simulink model "Takahashi1986_DTC"  (R2024b)
settings: Solver=FixedStepDiscrete  StartTime=0.0  StopTime=.62  FixedStep=Ts  RelTol=1e-3
InitFcn:
  | demoModel=bdroot; demoWorkspace=get_param(demoModel,'ModelWorkspace');
  | demoCases=getVariable(demoWorkspace,'DemoCases');
  | demoCaseName=get_param([demoModel '/Experiment_Settings'],'CaseName');
  | demoSelected=find(strcmp(demoCaseName,{demoCases.name}),1);
  | demoValues=demoCases(demoSelected).variables; demoNames=fieldnames(demoValues);
  | for demoIndex=1:numel(demoNames), assignin(demoWorkspace,demoNames{demoIndex},demoValues.(demoNames{demoIndex})); end
  | clear demoModel demoWorkspace demoCases demoCaseName demoSelected demoValues demoNames demoIndex;
model workspace (MAT data in the model file):
  DemoCases(1).name = 'Wide_band_0p40Nm'
  DemoCases(1).variables.ScenarioInput{1} = timeseries
  DemoCases(1).variables.ScenarioInput{1}.Name = 'unnamed'
  DemoCases(1).variables.ScenarioInput{1}.DataInfo = tsdata.datametadata
  DemoCases(1).variables.ScenarioInput{1}.DataInfo.Interpolation = tsdata.interpolation
  DemoCases(1).variables.ScenarioInput{1}.DataInfo.Interpolation.Fhandle : function handle (value not decoded)
  DemoCases(1).variables.ScenarioInput{1}.DataInfo.Interpolation.Name = 'linear'
  DemoCases(1).variables.ScenarioInput{1}.TimeInfo = tsdata.timemetadata
  DemoCases(1).variables.ScenarioInput{1}.TimeInfo.Length = 24801
  DemoCases(1).variables.ScenarioInput{1}.TimeInfo.DuplicateTimes = 0
  DemoCases(1).variables.ScenarioInput{1}.TimeInfo.Time_ = [0 2.5e-05 5e-05 7.5e-05 0.0001 0.000125 0.00015 0.000175 0.0002 0.000225 0.00025 0.000275 ... (24801 elements, 24801x1)]
  DemoCases(1).variables.ScenarioInput{1}.TimeInfo.Initialized = 1
  DemoCases(1).variables.ScenarioInput{1}.QualityInfo = tsdata.qualmetadata
  DemoCases(1).variables.ScenarioInput{1}.Data_ = [0.419999986887 0.419999986887 0.419999986887 0.419999986887 0.419999986887 0.419999986887 0.419999986887 0.419999986887 0.419999986887 0.419999986887 0.419999986887 0.419999986887 ... (24801 elements, 24801x1)]
  DemoCases(1).variables.ScenarioInput{2} = timeseries
  DemoCases(1).variables.ScenarioInput{2}.Name = 'unnamed'
  DemoCases(1).variables.ScenarioInput{2}.DataInfo = tsdata.datametadata
  DemoCases(1).variables.ScenarioInput{2}.DataInfo.Interpolation = tsdata.interpolation
  DemoCases(1).variables.ScenarioInput{2}.DataInfo.Interpolation.Fhandle : function handle (value not decoded)
  DemoCases(1).variables.ScenarioInput{2}.DataInfo.Interpolation.Name = 'linear'
  DemoCases(1).variables.ScenarioInput{2}.TimeInfo = tsdata.timemetadata
  DemoCases(1).variables.ScenarioInput{2}.TimeInfo.Length = 24801
  DemoCases(1).variables.ScenarioInput{2}.TimeInfo.DuplicateTimes = 0
  DemoCases(1).variables.ScenarioInput{2}.TimeInfo.Time_ = [0 2.5e-05 5e-05 7.5e-05 0.0001 0.000125 0.00015 0.000175 0.0002 0.000225 0.00025 0.000275 ... (24801 elements, 24801x1)]
  DemoCases(1).variables.ScenarioInput{2}.TimeInfo.Initialized = 1
  DemoCases(1).variables.ScenarioInput{2}.QualityInfo = tsdata.qualmetadata
  DemoCases(1).variables.ScenarioInput{2}.Data_ = [0 0 0 0 0 0 0 0 0 0 0 0 ... (24801 elements, 24801x1)]
  DemoCases(1).variables.ScenarioInput{3} = timeseries
  DemoCases(1).variables.ScenarioInput{3}.Name = 'unnamed'
  DemoCases(1).variables.ScenarioInput{3}.DataInfo = tsdata.datametadata
  DemoCases(1).variables.ScenarioInput{3}.DataInfo.Interpolation = tsdata.interpolation
  DemoCases(1).variables.ScenarioInput{3}.DataInfo.Interpolation.Fhandle : function handle (value not decoded)
  DemoCases(1).variables.ScenarioInput{3}.DataInfo.Interpolation.Name = 'linear'
  DemoCases(1).variables.ScenarioInput{3}.TimeInfo = tsdata.timemetadata
  DemoCases(1).variables.ScenarioInput{3}.TimeInfo.Length = 24801
  DemoCases(1).variables.ScenarioInput{3}.TimeInfo.DuplicateTimes = 0
  DemoCases(1).variables.ScenarioInput{3}.TimeInfo.Time_ = [0 2.5e-05 5e-05 7.5e-05 0.0001 0.000125 0.00015 0.000175 0.0002 0.000225 0.00025 0.000275 ... (24801 elements, 24801x1)]
  DemoCases(1).variables.ScenarioInput{3}.TimeInfo.Initialized = 1
  DemoCases(1).variables.ScenarioInput{3}.QualityInfo = tsdata.qualmetadata
  DemoCases(1).variables.ScenarioInput{3}.Data_ = [0.40000000596 0.40000000596 0.40000000596 0.40000000596 0.40000000596 0.40000000596 0.40000000596 0.40000000596 0.40000000596 0.40000000596 0.40000000596 0.40000000596 ... (24801 elements, 24801x1)]
  DemoCases(1).variables.ScenarioInput{4} = timeseries
  DemoCases(1).variables.ScenarioInput{4}.Name = 'unnamed'
  DemoCases(1).variables.ScenarioInput{4}.DataInfo = tsdata.datametadata
  DemoCases(1).variables.ScenarioInput{4}.DataInfo.Interpolation = tsdata.interpolation
  DemoCases(1).variables.ScenarioInput{4}.DataInfo.Interpolation.Fhandle : function handle (value not decoded)
  DemoCases(1).variables.ScenarioInput{4}.DataInfo.Interpolation.Name = 'linear'
  DemoCases(1).variables.ScenarioInput{4}.TimeInfo = tsdata.timemetadata
  DemoCases(1).variables.ScenarioInput{4}.TimeInfo.Length = 24801
  DemoCases(1).variables.ScenarioInput{4}.TimeInfo.DuplicateTimes = 0
  DemoCases(1).variables.ScenarioInput{4}.TimeInfo.Time_ = [0 2.5e-05 5e-05 7.5e-05 0.0001 0.000125 0.00015 0.000175 0.0002 0.000225 0.00025 0.000275 ... (24801 elements, 24801x1)]
  DemoCases(1).variables.ScenarioInput{4}.TimeInfo.Initialized = 1
  DemoCases(1).variables.ScenarioInput{4}.QualityInfo = tsdata.qualmetadata
  DemoCases(1).variables.ScenarioInput{4}.Data_ = [100 100 100 100 100 100 100 100 100 100 100 100 ... (24801 elements, 24801x1)]
  DemoCases(1).variables.ScenarioInput{5} = timeseries
  DemoCases(1).variables.ScenarioInput{5}.Name = 'unnamed'
  DemoCases(1).variables.ScenarioInput{5}.DataInfo = tsdata.datametadata
  DemoCases(1).variables.ScenarioInput{5}.DataInfo.Interpolation = tsdata.interpolation
  DemoCases(1).variables.ScenarioInput{5}.DataInfo.Interpolation.Fhandle : function handle (value not decoded)
  DemoCases(1).variables.ScenarioInput{5}.DataInfo.Interpolation.Name = 'linear'
  DemoCases(1).variables.ScenarioInput{5}.TimeInfo = tsdata.timemetadata
  DemoCases(1).variables.ScenarioInput{5}.TimeInfo.Length = 24801
  DemoCases(1).variables.ScenarioInput{5}.TimeInfo.DuplicateTimes = 0
  DemoCases(1).variables.ScenarioInput{5}.TimeInfo.Time_ = [0 2.5e-05 5e-05 7.5e-05 0.0001 0.000125 0.00015 0.000175 0.0002 0.000225 0.00025 0.000275 ... (24801 elements, 24801x1)]
  DemoCases(1).variables.ScenarioInput{5}.TimeInfo.Initialized = 1
  DemoCases(1).variables.ScenarioInput{5}.QualityInfo = tsdata.qualmetadata
  DemoCases(1).variables.ScenarioInput{5}.Data_ = [0 0 0 0 0 0 0 0 0 0 0 0 ... (24801 elements, 24801x1)]
  DemoCases(2).name = 'Narrow_band_0p15Nm'
  DemoCases(2).variables.ScenarioInput{1} = timeseries
  DemoCases(2).variables.ScenarioInput{1}.Name = 'unnamed'
  DemoCases(2).variables.ScenarioInput{1}.DataInfo = tsdata.datametadata
  DemoCases(2).variables.ScenarioInput{1}.DataInfo.Interpolation = tsdata.interpolation
  DemoCases(2).variables.ScenarioInput{1}.DataInfo.Interpolation.Fhandle : function handle (value not decoded)
  DemoCases(2).variables.ScenarioInput{1}.DataInfo.Interpolation.Name = 'linear'
  DemoCases(2).variables.ScenarioInput{1}.TimeInfo = tsdata.timemetadata
  DemoCases(2).variables.ScenarioInput{1}.TimeInfo.Length = 24801
  DemoCases(2).variables.ScenarioInput{1}.TimeInfo.DuplicateTimes = 0
  DemoCases(2).variables.ScenarioInput{1}.TimeInfo.Time_ = [0 2.5e-05 5e-05 7.5e-05 0.0001 0.000125 0.00015 0.000175 0.0002 0.000225 0.00025 0.000275 ... (24801 elements, 24801x1)]
  DemoCases(2).variables.ScenarioInput{1}.TimeInfo.Initialized = 1
  DemoCases(2).variables.ScenarioInput{1}.QualityInfo = tsdata.qualmetadata
  DemoCases(2).variables.ScenarioInput{1}.Data_ = [0.419999986887 0.419999986887 0.419999986887 0.419999986887 0.419999986887 0.419999986887 0.419999986887 0.419999986887 0.419999986887 0.419999986887 0.419999986887 0.419999986887 ... (24801 elements, 24801x1)]
  DemoCases(2).variables.ScenarioInput{2} = timeseries
  DemoCases(2).variables.ScenarioInput{2}.Name = 'unnamed'
  DemoCases(2).variables.ScenarioInput{2}.DataInfo = tsdata.datametadata
  DemoCases(2).variables.ScenarioInput{2}.DataInfo.Interpolation = tsdata.interpolation
  DemoCases(2).variables.ScenarioInput{2}.DataInfo.Interpolation.Fhandle : function handle (value not decoded)
  DemoCases(2).variables.ScenarioInput{2}.DataInfo.Interpolation.Name = 'linear'
  DemoCases(2).variables.ScenarioInput{2}.TimeInfo = tsdata.timemetadata
  DemoCases(2).variables.ScenarioInput{2}.TimeInfo.Length = 24801
  DemoCases(2).variables.ScenarioInput{2}.TimeInfo.DuplicateTimes = 0
  DemoCases(2).variables.ScenarioInput{2}.TimeInfo.Time_ = [0 2.5e-05 5e-05 7.5e-05 0.0001 0.000125 0.00015 0.000175 0.0002 0.000225 0.00025 0.000275 ... (24801 elements, 24801x1)]
  DemoCases(2).variables.ScenarioInput{2}.TimeInfo.Initialized = 1
  DemoCases(2).variables.ScenarioInput{2}.QualityInfo = tsdata.qualmetadata
  DemoCases(2).variables.ScenarioInput{2}.Data_ = [0 0 0 0 0 0 0 0 0 0 0 0 ... (24801 elements, 24801x1)]
  DemoCases(2).variables.ScenarioInput{3} = timeseries
  DemoCases(2).variables.ScenarioInput{3}.Name = 'unnamed'
  DemoCases(2).variables.ScenarioInput{3}.DataInfo = tsdata.datametadata
  DemoCases(2).variables.ScenarioInput{3}.DataInfo.Interpolation = tsdata.interpolation
  DemoCases(2).variables.ScenarioInput{3}.DataInfo.Interpolation.Fhandle : function handle (value not decoded)
  DemoCases(2).variables.ScenarioInput{3}.DataInfo.Interpolation.Name = 'linear'
  DemoCases(2).variables.ScenarioInput{3}.TimeInfo = tsdata.timemetadata
  DemoCases(2).variables.ScenarioInput{3}.TimeInfo.Length = 24801
  DemoCases(2).variables.ScenarioInput{3}.TimeInfo.DuplicateTimes = 0
  DemoCases(2).variables.ScenarioInput{3}.TimeInfo.Time_ = [0 2.5e-05 5e-05 7.5e-05 0.0001 0.000125 0.00015 0.000175 0.0002 0.000225 0.00025 0.000275 ... (24801 elements, 24801x1)]
  DemoCases(2).variables.ScenarioInput{3}.TimeInfo.Initialized = 1
  DemoCases(2).variables.ScenarioInput{3}.QualityInfo = tsdata.qualmetadata
  DemoCases(2).variables.ScenarioInput{3}.Data_ = [0.15000000596 0.15000000596 0.15000000596 0.15000000596 0.15000000596 0.15000000596 0.15000000596 0.15000000596 0.15000000596 0.15000000596 0.15000000596 0.15000000596 ... (24801 elements, 24801x1)]
  DemoCases(2).variables.ScenarioInput{4} = timeseries
  DemoCases(2).variables.ScenarioInput{4}.Name = 'unnamed'
  DemoCases(2).variables.ScenarioInput{4}.DataInfo = tsdata.datametadata
  DemoCases(2).variables.ScenarioInput{4}.DataInfo.Interpolation = tsdata.interpolation
  DemoCases(2).variables.ScenarioInput{4}.DataInfo.Interpolation.Fhandle : function handle (value not decoded)
  DemoCases(2).variables.ScenarioInput{4}.DataInfo.Interpolation.Name = 'linear'
  DemoCases(2).variables.ScenarioInput{4}.TimeInfo = tsdata.timemetadata
  DemoCases(2).variables.ScenarioInput{4}.TimeInfo.Length = 24801
  DemoCases(2).variables.ScenarioInput{4}.TimeInfo.DuplicateTimes = 0
  DemoCases(2).variables.ScenarioInput{4}.TimeInfo.Time_ = [0 2.5e-05 5e-05 7.5e-05 0.0001 0.000125 0.00015 0.000175 0.0002 0.000225 0.00025 0.000275 ... (24801 elements, 24801x1)]
  DemoCases(2).variables.ScenarioInput{4}.TimeInfo.Initialized = 1
  DemoCases(2).variables.ScenarioInput{4}.QualityInfo = tsdata.qualmetadata
  DemoCases(2).variables.ScenarioInput{4}.Data_ = [100 100 100 100 100 100 100 100 100 100 100 100 ... (24801 elements, 24801x1)]
  DemoCases(2).variables.ScenarioInput{5} = timeseries
  DemoCases(2).variables.ScenarioInput{5}.Name = 'unnamed'
  DemoCases(2).variables.ScenarioInput{5}.DataInfo = tsdata.datametadata
  DemoCases(2).variables.ScenarioInput{5}.DataInfo.Interpolation = tsdata.interpolation
  DemoCases(2).variables.ScenarioInput{5}.DataInfo.Interpolation.Fhandle : function handle (value not decoded)
  DemoCases(2).variables.ScenarioInput{5}.DataInfo.Interpolation.Name = 'linear'
  DemoCases(2).variables.ScenarioInput{5}.TimeInfo = tsdata.timemetadata
  DemoCases(2).variables.ScenarioInput{5}.TimeInfo.Length = 24801
  DemoCases(2).variables.ScenarioInput{5}.TimeInfo.DuplicateTimes = 0
  DemoCases(2).variables.ScenarioInput{5}.TimeInfo.Time_ = [0 2.5e-05 5e-05 7.5e-05 0.0001 0.000125 0.00015 0.000175 0.0002 0.000225 0.00025 0.000275 ... (24801 elements, 24801x1)]
  DemoCases(2).variables.ScenarioInput{5}.TimeInfo.Initialized = 1
  DemoCases(2).variables.ScenarioInput{5}.QualityInfo = tsdata.qualmetadata
  DemoCases(2).variables.ScenarioInput{5}.Data_ = [0 0 0 0 0 0 0 0 0 0 0 0 ... (24801 elements, 24801x1)]
  RecordedSignalNames = {'GateA'; 'GateB'; 'GateC'; 'FluxEstimate_Wb'; 'TorqueEstimate_Nm'; 'TorquePlant_Nm'; 'SpeedMechanical_radps'; 'Sector'; 'VectorIndex'; 'VAlpha_V'; 'VBeta_V'; 'IAlpha_A'; 'IBeta_A'}
  ScenarioInput{1} = timeseries
  ScenarioInput{1}.Name = 'unnamed'
  ScenarioInput{1}.DataInfo = tsdata.datametadata
  ScenarioInput{1}.DataInfo.Interpolation = tsdata.interpolation
  ScenarioInput{1}.DataInfo.Interpolation.Fhandle : function handle (value not decoded)
  ScenarioInput{1}.DataInfo.Interpolation.Name = 'linear'
  ScenarioInput{1}.TimeInfo = tsdata.timemetadata
  ScenarioInput{1}.TimeInfo.Length = 24801
  ScenarioInput{1}.TimeInfo.DuplicateTimes = 0
  ScenarioInput{1}.TimeInfo.Time_ = [0 2.5e-05 5e-05 7.5e-05 0.0001 0.000125 0.00015 0.000175 0.0002 0.000225 0.00025 0.000275 ... (24801 elements, 24801x1)]
  ScenarioInput{1}.TimeInfo.Initialized = 1
  ScenarioInput{1}.QualityInfo = tsdata.qualmetadata
  ScenarioInput{1}.Data_ = [0.419999986887 0.419999986887 0.419999986887 0.419999986887 0.419999986887 0.419999986887 0.419999986887 0.419999986887 0.419999986887 0.419999986887 0.419999986887 0.419999986887 ... (24801 elements, 24801x1)]
  ScenarioInput{2} = timeseries
  ScenarioInput{2}.Name = 'unnamed'
  ScenarioInput{2}.DataInfo = tsdata.datametadata
  ScenarioInput{2}.DataInfo.Interpolation = tsdata.interpolation
  ScenarioInput{2}.DataInfo.Interpolation.Fhandle : function handle (value not decoded)
  ScenarioInput{2}.DataInfo.Interpolation.Name = 'linear'
  ScenarioInput{2}.TimeInfo = tsdata.timemetadata
  ScenarioInput{2}.TimeInfo.Length = 24801
  ScenarioInput{2}.TimeInfo.DuplicateTimes = 0
  ScenarioInput{2}.TimeInfo.Time_ = [0 2.5e-05 5e-05 7.5e-05 0.0001 0.000125 0.00015 0.000175 0.0002 0.000225 0.00025 0.000275 ... (24801 elements, 24801x1)]
  ScenarioInput{2}.TimeInfo.Initialized = 1
  ScenarioInput{2}.QualityInfo = tsdata.qualmetadata
  ScenarioInput{2}.Data_ = [0 0 0 0 0 0 0 0 0 0 0 0 ... (24801 elements, 24801x1)]
  ScenarioInput{3} = timeseries
  ScenarioInput{3}.Name = 'unnamed'
  ScenarioInput{3}.DataInfo = tsdata.datametadata
  ScenarioInput{3}.DataInfo.Interpolation = tsdata.interpolation
  ScenarioInput{3}.DataInfo.Interpolation.Fhandle : function handle (value not decoded)
  ScenarioInput{3}.DataInfo.Interpolation.Name = 'linear'
  ScenarioInput{3}.TimeInfo = tsdata.timemetadata
  ScenarioInput{3}.TimeInfo.Length = 24801
  ScenarioInput{3}.TimeInfo.DuplicateTimes = 0
  ScenarioInput{3}.TimeInfo.Time_ = [0 2.5e-05 5e-05 7.5e-05 0.0001 0.000125 0.00015 0.000175 0.0002 0.000225 0.00025 0.000275 ... (24801 elements, 24801x1)]
  ScenarioInput{3}.TimeInfo.Initialized = 1
  ScenarioInput{3}.QualityInfo = tsdata.qualmetadata
  ScenarioInput{3}.Data_ = [0.15000000596 0.15000000596 0.15000000596 0.15000000596 0.15000000596 0.15000000596 0.15000000596 0.15000000596 0.15000000596 0.15000000596 0.15000000596 0.15000000596 ... (24801 elements, 24801x1)]
  ScenarioInput{4} = timeseries
  ScenarioInput{4}.Name = 'unnamed'
  ScenarioInput{4}.DataInfo = tsdata.datametadata
  ScenarioInput{4}.DataInfo.Interpolation = tsdata.interpolation
  ScenarioInput{4}.DataInfo.Interpolation.Fhandle : function handle (value not decoded)
  ScenarioInput{4}.DataInfo.Interpolation.Name = 'linear'
  ScenarioInput{4}.TimeInfo = tsdata.timemetadata
  ScenarioInput{4}.TimeInfo.Length = 24801
  ScenarioInput{4}.TimeInfo.DuplicateTimes = 0
  ScenarioInput{4}.TimeInfo.Time_ = [0 2.5e-05 5e-05 7.5e-05 0.0001 0.000125 0.00015 0.000175 0.0002 0.000225 0.00025 0.000275 ... (24801 elements, 24801x1)]
  ScenarioInput{4}.TimeInfo.Initialized = 1
  ScenarioInput{4}.QualityInfo = tsdata.qualmetadata
  ScenarioInput{4}.Data_ = [100 100 100 100 100 100 100 100 100 100 100 100 ... (24801 elements, 24801x1)]
  ScenarioInput{5} = timeseries
  ScenarioInput{5}.Name = 'unnamed'
  ScenarioInput{5}.DataInfo = tsdata.datametadata
  ScenarioInput{5}.DataInfo.Interpolation = tsdata.interpolation
  ScenarioInput{5}.DataInfo.Interpolation.Fhandle : function handle (value not decoded)
  ScenarioInput{5}.DataInfo.Interpolation.Name = 'linear'
  ScenarioInput{5}.TimeInfo = tsdata.timemetadata
  ScenarioInput{5}.TimeInfo.Length = 24801
  ScenarioInput{5}.TimeInfo.DuplicateTimes = 0
  ScenarioInput{5}.TimeInfo.Time_ = [0 2.5e-05 5e-05 7.5e-05 0.0001 0.000125 0.00015 0.000175 0.0002 0.000225 0.00025 0.000275 ... (24801 elements, 24801x1)]
  ScenarioInput{5}.TimeInfo.Initialized = 1
  ScenarioInput{5}.QualityInfo = tsdata.qualmetadata
  ScenarioInput{5}.Data_ = [0 0 0 0 0 0 0 0 0 0 0 0 ... (24801 elements, 24801x1)]
values from neighbouring files (symbols this model uses):
  Bshaft = 0.0045    [Takahashi1986_DTC.sldd]
  FluxBand = 0.008    [Takahashi1986_DTC.sldd]
  Jshaft = 0.028    [Takahashi1986_DTC.sldd]
  Lm = 0.088    [Takahashi1986_DTC.sldd]
  Lr = 0.094    [Takahashi1986_DTC.sldd]
  Ls = 0.094    [Takahashi1986_DTC.sldd]
  PolePairs = 2.0    [Takahashi1986_DTC.sldd]
  Rr = 0.62    [Takahashi1986_DTC.sldd]
  Rs = 0.82    [Takahashi1986_DTC.sldd]
  Ts = 2.5E-5    [Takahashi1986_DTC.sldd]
settings Model: DataDictionary=Takahashi1986_DTC.sldd  Creator=lxy  LastModifiedBy=lxy

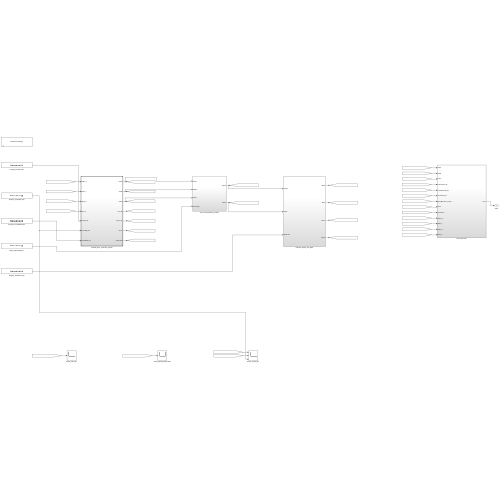
[thumbnail: Simulink's stored preview of the top-level diagram]
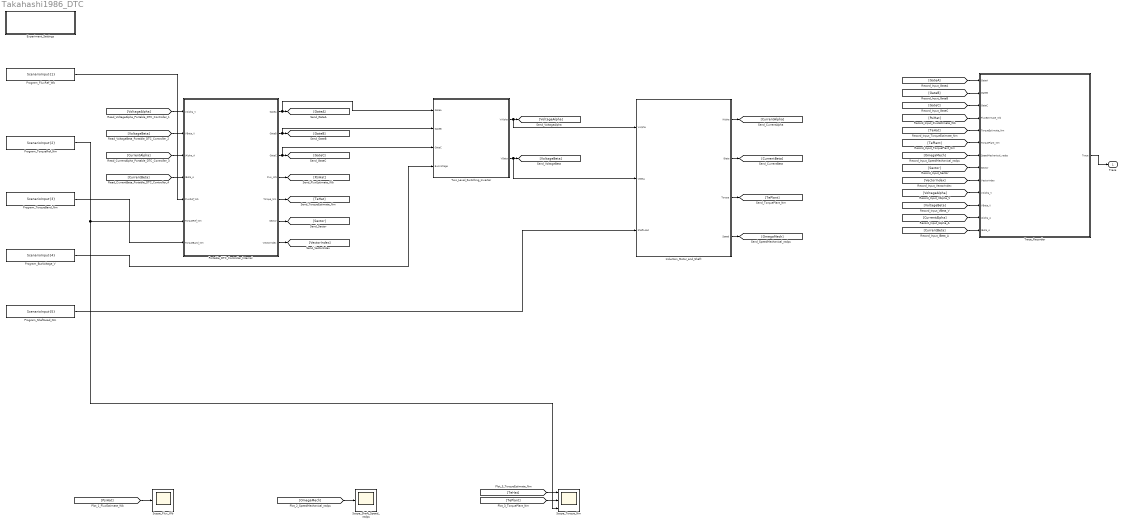
== system Takahashi1986_DTC ==
  Experiment_Settings : Subsystem  mask{CaseName=Narrow_band_0p15Nm}
      mask prompts: CaseName "Experiment"
      mask help: Select the experiment, then click Run. Parameters and test inputs are included in the download.
      mask TypeOptions CaseName: Wide_band_0p40Nm | Narrow_band_0p15Nm
      mask Display: disp('Experiment settings')
  Induction_Motor_and_Shaft : Subsystem
  Portable_DTC_Controller_Internal : Subsystem  TreatAsAtomicUnit=on
  Program_BusVoltage_V : FromWorkspace  VariableName=ScenarioInput{4}  SampleTime=Ts  Interpolate=off  OutputAfterFinalValue=Holding final value
  Program_FluxRef_Wb : FromWorkspace  VariableName=ScenarioInput{1}  SampleTime=Ts  Interpolate=off  OutputAfterFinalValue=Holding final value
  Program_ShaftLoad_Nm : FromWorkspace  VariableName=ScenarioInput{5}  SampleTime=Ts  Interpolate=off  OutputAfterFinalValue=Holding final value
  Program_TorqueBand_Nm : FromWorkspace  VariableName=ScenarioInput{3}  SampleTime=Ts  Interpolate=off  OutputAfterFinalValue=Holding final value
  Program_TorqueRef_Nm : FromWorkspace  VariableName=ScenarioInput{2}  SampleTime=Ts  Interpolate=off  OutputAfterFinalValue=Holding final value
  Scope_Flux_Wb : Scope
  Scope_Shaft_Speed_radps : Scope
  Scope_Torque_Nm : Scope  NumInputPorts=3
  Trace_Recorder : Subsystem
  Two_Level_Switching_Inverter : Subsystem
  Trace : Outport
  wires:
  Portable_DTC_Controller_Internal/7(VectorIndex) -> [VectorIndex]
  Portable_DTC_Controller_Internal/6(Sector) -> [Sector]
  Portable_DTC_Controller_Internal/5(Torque_Nm) -> [TeHat]
  Portable_DTC_Controller_Internal/4(Flux_Wb) -> [PsiHat]
  Portable_DTC_Controller_Internal/3(GateC) -> [GateC], Two_Level_Switching_Inverter/3(GateC)
  Portable_DTC_Controller_Internal/2(GateB) -> [GateB], Two_Level_Switching_Inverter/2(GateB)
  Portable_DTC_Controller_Internal/1(GateA) -> Two_Level_Switching_Inverter/1(GateA), [GateA]
  [CurrentBeta] -> Portable_DTC_Controller_Internal/4(IBeta_A)
  [CurrentAlpha] -> Portable_DTC_Controller_Internal/3(IAlpha_A)
  [VoltageBeta] -> Portable_DTC_Controller_Internal/2(VBeta_V)
  [VoltageAlpha] -> Portable_DTC_Controller_Internal/1(VAlpha_V)
  Program_FluxRef_Wb/1 -> Portable_DTC_Controller_Internal/5(FluxRef_Wb)
  Program_TorqueBand_Nm/1 -> Portable_DTC_Controller_Internal/7(TorqueBand_Nm)
  Program_BusVoltage_V/1 -> Two_Level_Switching_Inverter/4(BusVoltage)
  Program_ShaftLoad_Nm/1 -> Induction_Motor_and_Shaft/3(ShaftLoad)
  Two_Level_Switching_Inverter/2(VBeta) -> Induction_Motor_and_Shaft/2(VBeta), [VoltageBeta]
  Two_Level_Switching_Inverter/1(VAlpha) -> Induction_Motor_and_Shaft/1(VAlpha), [VoltageAlpha]
  Induction_Motor_and_Shaft/1(IAlpha) -> [CurrentAlpha]
  Induction_Motor_and_Shaft/2(IBeta) -> [CurrentBeta]
  Induction_Motor_and_Shaft/3(Torque) -> [TePlant]
  Induction_Motor_and_Shaft/4(Speed) -> [OmegaMech]
  [CurrentBeta] -> Trace_Recorder/13(IBeta_A)
  [CurrentAlpha] -> Trace_Recorder/12(IAlpha_A)
  [VoltageBeta] -> Trace_Recorder/11(VBeta_V)
  [VoltageAlpha] -> Trace_Recorder/10(VAlpha_V)
  [VectorIndex] -> Trace_Recorder/9(VectorIndex)
  [Sector] -> Trace_Recorder/8(Sector)
  [OmegaMech] -> Trace_Recorder/7(SpeedMechanical_radps)
  [TePlant] -> Trace_Recorder/6(TorquePlant_Nm)
  [TeHat] -> Trace_Recorder/5(TorqueEstimate_Nm)
  [PsiHat] -> Trace_Recorder/4(FluxEstimate_Wb)
  [GateC] -> Trace_Recorder/3(GateC)
  [GateB] -> Trace_Recorder/2(GateB)
  [GateA] -> Trace_Recorder/1(GateA)
  Trace_Recorder/1(Trace) -> Trace/1
  [TePlant] -> Scope_Torque_Nm/2
  [TeHat] -> Scope_Torque_Nm/1
  [OmegaMech] -> Scope_Shaft_Speed_radps/1
  [PsiHat] -> Scope_Flux_Wb/1
  Program_TorqueRef_Nm/1 -> Scope_Torque_Nm/3, Portable_DTC_Controller_Internal/6(TorqueRef_Nm)

== system Takahashi1986_DTC/Experiment_Settings ==

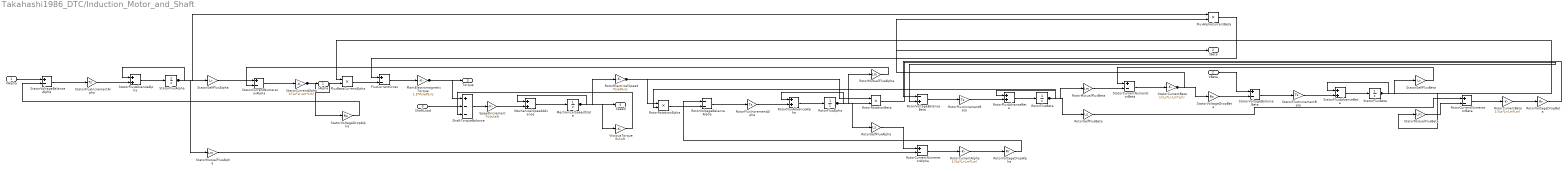
== system Takahashi1986_DTC/Induction_Motor_and_Shaft ==
  VAlpha : Inport
  VBeta : Inport  Port=2
  ShaftLoad : Inport  Port=3
  FluxAlphaCurrentBeta : Product  Inputs=**
  FluxBetaCurrentAlpha : Product  Inputs=**
  FluxCurrentCross : Sum  Inputs=+-
  MechanicalSpeedAdvance : Sum
  MechanicalSpeedState : UnitDelay  SampleTime=Ts  HasFrameUpgradeWarning=on
  PlantElectromagneticTorque : Gain  Gain=1.5*PolePairs
  RotorCurrentAlpha : Gain  Gain=1/(Ls*Lr-Lm*Lm)
  RotorCurrentBeta : Gain  Gain=1/(Ls*Lr-Lm*Lm)
  RotorCurrentNumeratorAlpha : Sum  Inputs=+-
  RotorCurrentNumeratorBeta : Sum  Inputs=+-
  RotorElectricalSpeed : Gain  Gain=PolePairs
  RotorFluxAdvanceAlpha : Sum
  RotorFluxAdvanceBeta : Sum
  RotorFluxAlpha : UnitDelay  SampleTime=Ts  HasFrameUpgradeWarning=on
  RotorFluxBeta : UnitDelay  SampleTime=Ts  HasFrameUpgradeWarning=on
  RotorFluxIncrementAlpha : Gain  Gain=Ts
  RotorFluxIncrementBeta : Gain  Gain=Ts
  RotorMutualFluxAlpha : Gain  Gain=Lm
  RotorMutualFluxBeta : Gain  Gain=Lm
  RotorRotationAlpha : Product  Inputs=**
  RotorRotationBeta : Product  Inputs=**
  RotorSelfFluxAlpha : Gain  Gain=Ls
  RotorSelfFluxBeta : Gain  Gain=Ls
  RotorVoltageBalanceAlpha : Sum  Inputs=--
  RotorVoltageBalanceBeta : Sum  Inputs=-+
  RotorVoltageDropAlpha : Gain  Gain=Rr
  RotorVoltageDropBeta : Gain  Gain=Rr
  ShaftTorqueBalance : Sum  Inputs=+--
  SpeedIncrement : Gain  Gain=Ts/Jshaft
  StatorCurrentAlpha : Gain  Gain=1/(Ls*Lr-Lm*Lm)
  StatorCurrentBeta : Gain  Gain=1/(Ls*Lr-Lm*Lm)
  StatorCurrentNumeratorAlpha : Sum  Inputs=+-
  StatorCurrentNumeratorBeta : Sum  Inputs=+-
  StatorFluxAdvanceAlpha : Sum
  StatorFluxAdvanceBeta : Sum
  StatorFluxAlpha : UnitDelay  SampleTime=Ts  HasFrameUpgradeWarning=on
  StatorFluxBeta : UnitDelay  SampleTime=Ts  HasFrameUpgradeWarning=on
  StatorFluxIncrementAlpha : Gain  Gain=Ts
  StatorFluxIncrementBeta : Gain  Gain=Ts
  StatorMutualFluxAlpha : Gain  Gain=Lm
  StatorMutualFluxBeta : Gain  Gain=Lm
  StatorSelfFluxAlpha : Gain  Gain=Lr
  StatorSelfFluxBeta : Gain  Gain=Lr
  StatorVoltageBalanceAlpha : Sum  Inputs=+-
  StatorVoltageBalanceBeta : Sum  Inputs=+-
  StatorVoltageDropAlpha : Gain  Gain=Rs
  StatorVoltageDropBeta : Gain  Gain=Rs
  ViscousTorque : Gain  Gain=Bshaft
  IAlpha : Outport
  IBeta : Outport  Port=2
  Torque : Outport  Port=3
  Speed : Outport  Port=4
  wires:
  MechanicalSpeedAdvance/1 -> MechanicalSpeedState/1
  SpeedIncrement/1 -> MechanicalSpeedAdvance/2
  ShaftTorqueBalance/1 -> SpeedIncrement/1
  ViscousTorque/1 -> ShaftTorqueBalance/3
  ShaftLoad/1 -> ShaftTorqueBalance/2
  PlantElectromagneticTorque/1 -> Torque/1, ShaftTorqueBalance/1
  FluxCurrentCross/1 -> PlantElectromagneticTorque/1
  FluxBetaCurrentAlpha/1 -> FluxCurrentCross/2
  FluxAlphaCurrentBeta/1 -> FluxCurrentCross/1
  RotorFluxAdvanceBeta/1 -> RotorFluxBeta/1
  RotorFluxIncrementBeta/1 -> RotorFluxAdvanceBeta/2
  RotorVoltageBalanceBeta/1 -> RotorFluxIncrementBeta/1
  StatorFluxAdvanceBeta/1 -> StatorFluxBeta/1
  StatorFluxIncrementBeta/1 -> StatorFluxAdvanceBeta/2
  StatorVoltageBalanceBeta/1 -> StatorFluxIncrementBeta/1
  RotorRotationBeta/1 -> RotorVoltageBalanceBeta/2
  RotorVoltageDropBeta/1 -> RotorVoltageBalanceBeta/1
  RotorCurrentBeta/1 -> RotorVoltageDropBeta/1
  StatorVoltageDropBeta/1 -> StatorVoltageBalanceBeta/2
  VBeta/1 -> StatorVoltageBalanceBeta/1
  StatorCurrentBeta/1 -> StatorVoltageDropBeta/1, IBeta/1, FluxAlphaCurrentBeta/2
  RotorCurrentNumeratorBeta/1 -> RotorCurrentBeta/1
  StatorMutualFluxBeta/1 -> RotorCurrentNumeratorBeta/2
  RotorSelfFluxBeta/1 -> RotorCurrentNumeratorBeta/1
  StatorCurrentNumeratorBeta/1 -> StatorCurrentBeta/1
  RotorMutualFluxBeta/1 -> StatorCurrentNumeratorBeta/2
  StatorSelfFluxBeta/1 -> StatorCurrentNumeratorBeta/1
  StatorFluxBeta/1 -> StatorMutualFluxBeta/1, StatorFluxAdvanceBeta/1, StatorSelfFluxBeta/1, FluxBetaCurrentAlpha/1
  RotorFluxAdvanceAlpha/1 -> RotorFluxAlpha/1
  RotorFluxIncrementAlpha/1 -> RotorFluxAdvanceAlpha/2
  RotorVoltageBalanceAlpha/1 -> RotorFluxIncrementAlpha/1
  StatorFluxAdvanceAlpha/1 -> StatorFluxAlpha/1
  StatorFluxIncrementAlpha/1 -> StatorFluxAdvanceAlpha/2
  StatorVoltageBalanceAlpha/1 -> StatorFluxIncrementAlpha/1
  RotorRotationAlpha/1 -> RotorVoltageBalanceAlpha/2
  RotorVoltageDropAlpha/1 -> RotorVoltageBalanceAlpha/1
  RotorFluxBeta/1 -> RotorRotationAlpha/2, RotorMutualFluxBeta/1, RotorSelfFluxBeta/1, RotorFluxAdvanceBeta/1
  RotorElectricalSpeed/1 -> RotorRotationAlpha/1, RotorRotationBeta/1
  RotorCurrentAlpha/1 -> RotorVoltageDropAlpha/1
  StatorVoltageDropAlpha/1 -> StatorVoltageBalanceAlpha/2
  VAlpha/1 -> StatorVoltageBalanceAlpha/1
  StatorCurrentAlpha/1 -> StatorVoltageDropAlpha/1, IAlpha/1, FluxBetaCurrentAlpha/2
  RotorCurrentNumeratorAlpha/1 -> RotorCurrentAlpha/1
  StatorMutualFluxAlpha/1 -> RotorCurrentNumeratorAlpha/2
  RotorSelfFluxAlpha/1 -> RotorCurrentNumeratorAlpha/1
  StatorCurrentNumeratorAlpha/1 -> StatorCurrentAlpha/1
  RotorMutualFluxAlpha/1 -> StatorCurrentNumeratorAlpha/2
  StatorSelfFluxAlpha/1 -> StatorCurrentNumeratorAlpha/1
  RotorFluxAlpha/1 -> RotorMutualFluxAlpha/1, RotorSelfFluxAlpha/1, RotorFluxAdvanceAlpha/1, RotorRotationBeta/2
  StatorFluxAlpha/1 -> StatorSelfFluxAlpha/1, StatorFluxAdvanceAlpha/1, StatorMutualFluxAlpha/1, FluxAlphaCurrentBeta/1
  MechanicalSpeedState/1 -> RotorElectricalSpeed/1, ViscousTorque/1, MechanicalSpeedAdvance/1, Speed/1

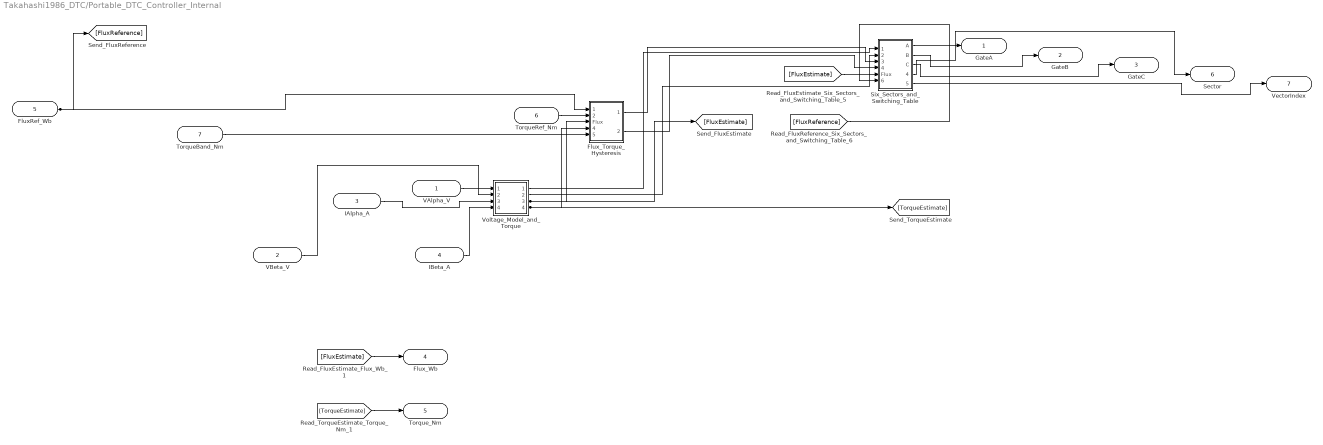
== system Takahashi1986_DTC/Portable_DTC_Controller_Internal ==
  VAlpha_V : Inport  OutDataTypeStr=single  SampleTime=Ts
  VBeta_V : Inport  Port=2  OutDataTypeStr=single  SampleTime=Ts
  IAlpha_A : Inport  Port=3  OutDataTypeStr=single  SampleTime=Ts
  IBeta_A : Inport  Port=4  OutDataTypeStr=single  SampleTime=Ts
  FluxRef_Wb : Inport  Port=5  OutDataTypeStr=single  SampleTime=Ts
  TorqueRef_Nm : Inport  Port=6  OutDataTypeStr=single  SampleTime=Ts
  TorqueBand_Nm : Inport  Port=7  OutDataTypeStr=single  SampleTime=Ts
  Flux_Torque_Hysteresis : Subsystem
  Six_Sectors_and_Switching_Table : Subsystem
  Voltage_Model_and_Torque : Subsystem
  GateA : Outport
  GateB : Outport  Port=2
  GateC : Outport  Port=3
  Flux_Wb : Outport  Port=4
  Torque_Nm : Outport  Port=5
  Sector : Outport  Port=6
  VectorIndex : Outport  Port=7
  wires:
  VAlpha_V/1 -> Voltage_Model_and_Torque/1(VAlpha)
  VBeta_V/1 -> Voltage_Model_and_Torque/2(VBeta)
  IAlpha_A/1 -> Voltage_Model_and_Torque/3(IAlpha)
  IBeta_A/1 -> Voltage_Model_and_Torque/4(IBeta)
  FluxRef_Wb/1 -> [FluxReference], Flux_Torque_Hysteresis/1(FluxRef)
  TorqueRef_Nm/1 -> Flux_Torque_Hysteresis/2(TorqueRef)
  Voltage_Model_and_Torque/3(FluxMagnitude) -> Flux_Torque_Hysteresis/3(Flux), [FluxEstimate]
  Voltage_Model_and_Torque/4(TorqueEstimate) -> Flux_Torque_Hysteresis/4(Torque), [TorqueEstimate]
  TorqueBand_Nm/1 -> Flux_Torque_Hysteresis/5(TorqueBand)
  Voltage_Model_and_Torque/1(FluxAlpha) -> Six_Sectors_and_Switching_Table/1(Alpha)
  Voltage_Model_and_Torque/2(FluxBeta) -> Six_Sectors_and_Switching_Table/2(Beta)
  Flux_Torque_Hysteresis/1(FluxFlag) -> Six_Sectors_and_Switching_Table/3(FluxFlag)
  Flux_Torque_Hysteresis/2(TorqueFlag) -> Six_Sectors_and_Switching_Table/4(TorqueFlag)
  Six_Sectors_and_Switching_Table/1(A) -> GateA/1
  Six_Sectors_and_Switching_Table/2(B) -> GateB/1
  Six_Sectors_and_Switching_Table/3(C) -> GateC/1
  Six_Sectors_and_Switching_Table/4(SectorNumber) -> Sector/1
  Six_Sectors_and_Switching_Table/5(Index) -> VectorIndex/1
  [FluxReference] -> Six_Sectors_and_Switching_Table/6(FluxRef)
  [FluxEstimate] -> Six_Sectors_and_Switching_Table/5(Flux)
  [FluxEstimate] -> Flux_Wb/1
  [TorqueEstimate] -> Torque_Nm/1

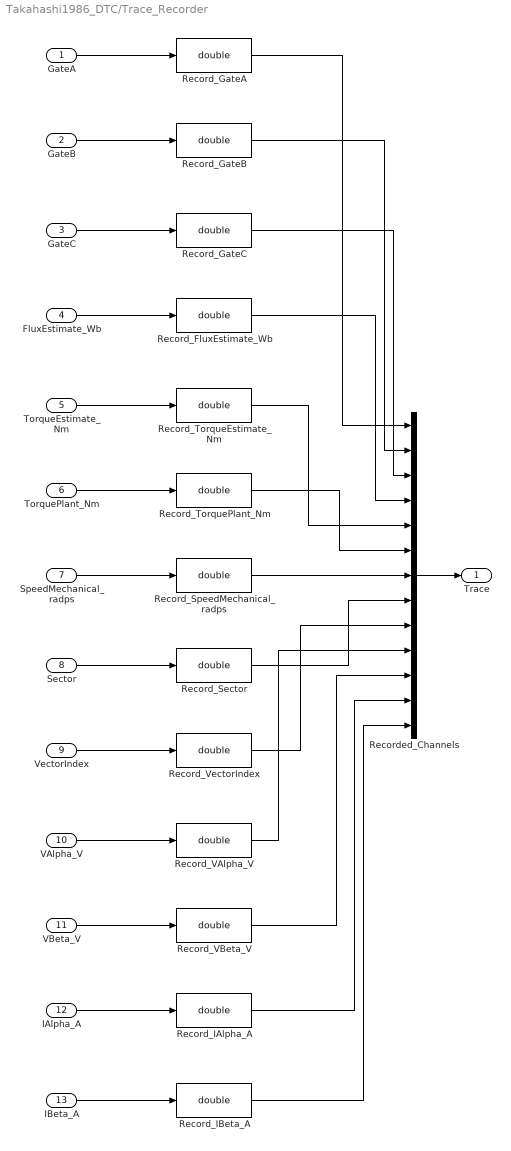
== system Takahashi1986_DTC/Trace_Recorder ==
  GateA : Inport
  GateB : Inport  Port=2
  GateC : Inport  Port=3
  FluxEstimate_Wb : Inport  Port=4
  TorqueEstimate_Nm : Inport  Port=5
  TorquePlant_Nm : Inport  Port=6
  SpeedMechanical_radps : Inport  Port=7
  Sector : Inport  Port=8
  VectorIndex : Inport  Port=9
  VAlpha_V : Inport  Port=10
  VBeta_V : Inport  Port=11
  IAlpha_A : Inport  Port=12
  IBeta_A : Inport  Port=13
  Record_FluxEstimate_Wb : DataTypeConversion  OutDataTypeStr=double  SaturateOnIntegerOverflow=off  RndMeth=Floor
  Record_GateA : DataTypeConversion  OutDataTypeStr=double  SaturateOnIntegerOverflow=off  RndMeth=Floor
  Record_GateB : DataTypeConversion  OutDataTypeStr=double  SaturateOnIntegerOverflow=off  RndMeth=Floor
  Record_GateC : DataTypeConversion  OutDataTypeStr=double  SaturateOnIntegerOverflow=off  RndMeth=Floor
  Record_IAlpha_A : DataTypeConversion  OutDataTypeStr=double  SaturateOnIntegerOverflow=off  RndMeth=Floor
  Record_IBeta_A : DataTypeConversion  OutDataTypeStr=double  SaturateOnIntegerOverflow=off  RndMeth=Floor
  Record_Sector : DataTypeConversion  OutDataTypeStr=double  SaturateOnIntegerOverflow=off  RndMeth=Floor
  Record_SpeedMechanical_radps : DataTypeConversion  OutDataTypeStr=double  SaturateOnIntegerOverflow=off  RndMeth=Floor
  Record_TorqueEstimate_Nm : DataTypeConversion  OutDataTypeStr=double  SaturateOnIntegerOverflow=off  RndMeth=Floor
  Record_TorquePlant_Nm : DataTypeConversion  OutDataTypeStr=double  SaturateOnIntegerOverflow=off  RndMeth=Floor
  Record_VAlpha_V : DataTypeConversion  OutDataTypeStr=double  SaturateOnIntegerOverflow=off  RndMeth=Floor
  Record_VBeta_V : DataTypeConversion  OutDataTypeStr=double  SaturateOnIntegerOverflow=off  RndMeth=Floor
  Record_VectorIndex : DataTypeConversion  OutDataTypeStr=double  SaturateOnIntegerOverflow=off  RndMeth=Floor
  Recorded_Channels : Mux  Inputs=13
  Trace : Outport
  wires:
  Recorded_Channels/1 -> Trace/1
  Record_IBeta_A/1 -> Recorded_Channels/13
  IBeta_A/1 -> Record_IBeta_A/1
  Record_IAlpha_A/1 -> Recorded_Channels/12
  IAlpha_A/1 -> Record_IAlpha_A/1
  Record_VBeta_V/1 -> Recorded_Channels/11
  VBeta_V/1 -> Record_VBeta_V/1
  Record_VAlpha_V/1 -> Recorded_Channels/10
  VAlpha_V/1 -> Record_VAlpha_V/1
  Record_VectorIndex/1 -> Recorded_Channels/9
  VectorIndex/1 -> Record_VectorIndex/1
  Record_Sector/1 -> Recorded_Channels/8
  Sector/1 -> Record_Sector/1
  Record_SpeedMechanical_radps/1 -> Recorded_Channels/7
  SpeedMechanical_radps/1 -> Record_SpeedMechanical_radps/1
  Record_TorquePlant_Nm/1 -> Recorded_Channels/6
  TorquePlant_Nm/1 -> Record_TorquePlant_Nm/1
  Record_TorqueEstimate_Nm/1 -> Recorded_Channels/5
  TorqueEstimate_Nm/1 -> Record_TorqueEstimate_Nm/1
  Record_FluxEstimate_Wb/1 -> Recorded_Channels/4
  FluxEstimate_Wb/1 -> Record_FluxEstimate_Wb/1
  Record_GateC/1 -> Recorded_Channels/3
  GateC/1 -> Record_GateC/1
  Record_GateB/1 -> Recorded_Channels/2
  GateB/1 -> Record_GateB/1
  Record_GateA/1 -> Recorded_Channels/1
  GateA/1 -> Record_GateA/1

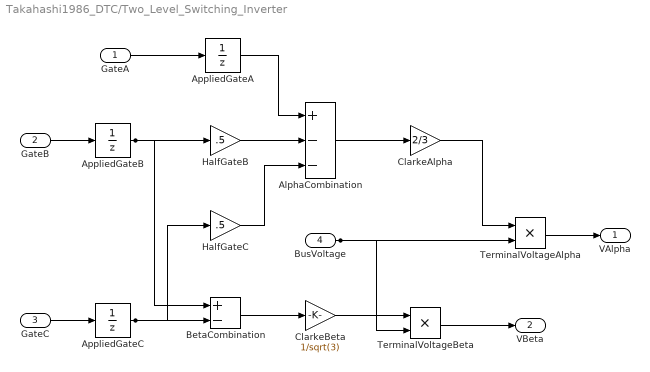
== system Takahashi1986_DTC/Two_Level_Switching_Inverter ==
  GateA : Inport
  GateB : Inport  Port=2
  GateC : Inport  Port=3
  BusVoltage : Inport  Port=4
  AlphaCombination : Sum  Inputs=+--
  AppliedGateA : UnitDelay  SampleTime=Ts  HasFrameUpgradeWarning=on
  AppliedGateB : UnitDelay  SampleTime=Ts  HasFrameUpgradeWarning=on
  AppliedGateC : UnitDelay  SampleTime=Ts  HasFrameUpgradeWarning=on
  BetaCombination : Sum  Inputs=+-
  ClarkeAlpha : Gain  Gain=2/3
  ClarkeBeta : Gain  Gain=1/sqrt(3)
  HalfGateB : Gain  Gain=.5
  HalfGateC : Gain  Gain=.5
  TerminalVoltageAlpha : Product  Inputs=**
  TerminalVoltageBeta : Product  Inputs=**
  VAlpha : Outport
  VBeta : Outport  Port=2
  wires:
  TerminalVoltageBeta/1 -> VBeta/1
  ClarkeBeta/1 -> TerminalVoltageBeta/1
  TerminalVoltageAlpha/1 -> VAlpha/1
  BusVoltage/1 -> TerminalVoltageAlpha/2, TerminalVoltageBeta/2
  ClarkeAlpha/1 -> TerminalVoltageAlpha/1
  BetaCombination/1 -> ClarkeBeta/1
  AlphaCombination/1 -> ClarkeAlpha/1
  HalfGateC/1 -> AlphaCombination/3
  HalfGateB/1 -> AlphaCombination/2
  AppliedGateA/1 -> AlphaCombination/1
  AppliedGateC/1 -> HalfGateC/1, BetaCombination/2
  AppliedGateB/1 -> HalfGateB/1, BetaCombination/1
  GateC/1 -> AppliedGateC/1
  GateB/1 -> AppliedGateB/1
  GateA/1 -> AppliedGateA/1

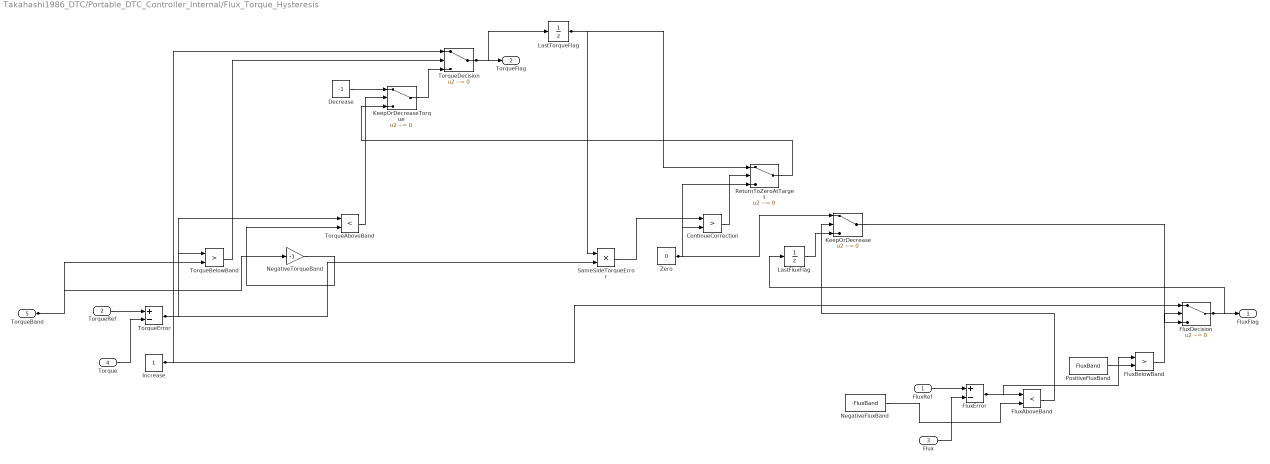
== system Takahashi1986_DTC/Portable_DTC_Controller_Internal/Flux_Torque_Hysteresis ==
  FluxRef : Inport
  TorqueRef : Inport  Port=2
  Flux : Inport  Port=3
  Torque : Inport  Port=4
  TorqueBand : Inport  Port=5
  ContinueCorrection : RelationalOperator  Operator=>  OutDataTypeStr=boolean  RndMeth=Simplest  InputSameDT=off
  Decrease : Constant  Value=-1  OutDataTypeStr=single
  FluxAboveBand : RelationalOperator  Operator=<  OutDataTypeStr=boolean  RndMeth=Simplest  InputSameDT=off
  FluxBelowBand : RelationalOperator  Operator=>  OutDataTypeStr=boolean  RndMeth=Simplest  InputSameDT=off
  FluxDecision : Switch  Criteria=u2 ~= 0  SaturateOnIntegerOverflow=off  InputSameDT=off
  FluxError : Sum  Inputs=+-
  Increase : Constant  OutDataTypeStr=single
  KeepOrDecrease : Switch  Criteria=u2 ~= 0  SaturateOnIntegerOverflow=off  InputSameDT=off
  KeepOrDecreaseTorque : Switch  Criteria=u2 ~= 0  SaturateOnIntegerOverflow=off  InputSameDT=off
  LastFluxFlag : UnitDelay  InitialCondition=1  SampleTime=Ts  HasFrameUpgradeWarning=on
  LastTorqueFlag : UnitDelay  SampleTime=Ts  HasFrameUpgradeWarning=on
  NegativeFluxBand : Constant  Value=-FluxBand  OutDataTypeStr=single
  NegativeTorqueBand : Gain  Gain=-1
  PositiveFluxBand : Constant  Value=FluxBand  OutDataTypeStr=single
  ReturnToZeroAtTarget : Switch  Criteria=u2 ~= 0  SaturateOnIntegerOverflow=off  InputSameDT=off
  SameSideTorqueError : Product  Inputs=**
  TorqueAboveBand : RelationalOperator  Operator=<  OutDataTypeStr=boolean  RndMeth=Simplest  InputSameDT=off
  TorqueBelowBand : RelationalOperator  Operator=>  OutDataTypeStr=boolean  RndMeth=Simplest  InputSameDT=off
  TorqueDecision : Switch  Criteria=u2 ~= 0  SaturateOnIntegerOverflow=off  InputSameDT=off
  TorqueError : Sum  Inputs=+-
  Zero : Constant  Value=0  OutDataTypeStr=single
  FluxFlag : Outport
  TorqueFlag : Outport  Port=2
  wires:
  TorqueDecision/1 -> LastTorqueFlag/1, TorqueFlag/1
  KeepOrDecreaseTorque/1 -> TorqueDecision/3
  TorqueBelowBand/1 -> TorqueDecision/2
  ReturnToZeroAtTarget/1 -> KeepOrDecreaseTorque/3
  TorqueAboveBand/1 -> KeepOrDecreaseTorque/2
  Decrease/1 -> KeepOrDecreaseTorque/1
  ContinueCorrection/1 -> ReturnToZeroAtTarget/2
  SameSideTorqueError/1 -> ContinueCorrection/1
  LastTorqueFlag/1 -> SameSideTorqueError/1, ReturnToZeroAtTarget/1
  NegativeTorqueBand/1 -> TorqueAboveBand/2
  TorqueError/1 -> SameSideTorqueError/2, TorqueBelowBand/1, TorqueAboveBand/1
  Torque/1 -> TorqueError/2
  TorqueRef/1 -> TorqueError/1
  FluxDecision/1 -> LastFluxFlag/1, FluxFlag/1
  KeepOrDecrease/1 -> FluxDecision/3
  FluxBelowBand/1 -> FluxDecision/2
  Increase/1 -> FluxDecision/1, TorqueDecision/1
  LastFluxFlag/1 -> KeepOrDecrease/3
  FluxAboveBand/1 -> KeepOrDecrease/2
  Zero/1 -> KeepOrDecrease/1, ContinueCorrection/2, ReturnToZeroAtTarget/3
  NegativeFluxBand/1 -> FluxAboveBand/2
  PositiveFluxBand/1 -> FluxBelowBand/2
  FluxError/1 -> FluxBelowBand/1, FluxAboveBand/1
  TorqueBand/1 -> TorqueBelowBand/2, NegativeTorqueBand/1
  Flux/1 -> FluxError/2
  FluxRef/1 -> FluxError/1

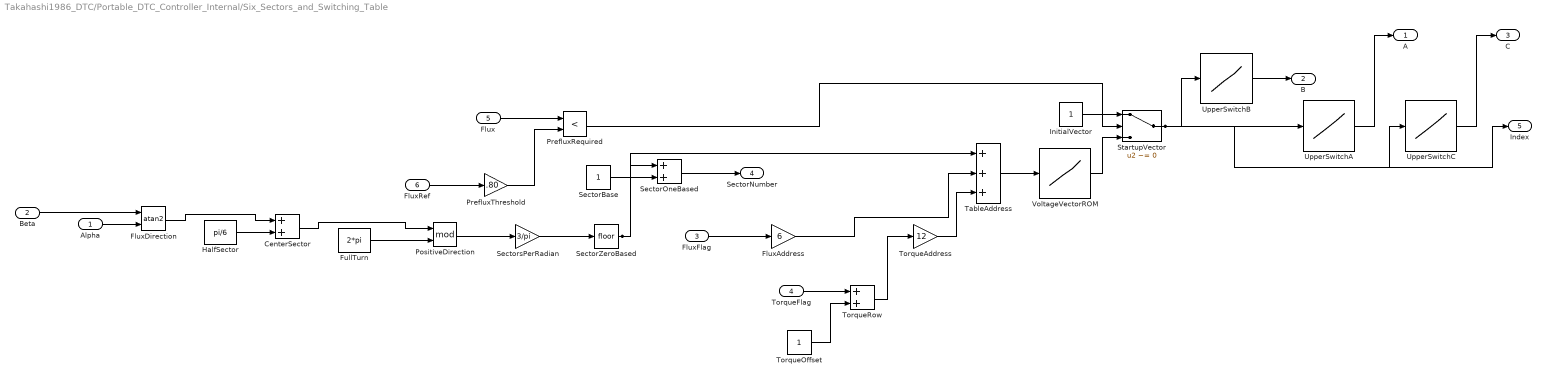
== system Takahashi1986_DTC/Portable_DTC_Controller_Internal/Six_Sectors_and_Switching_Table ==
  Alpha : Inport
  Beta : Inport  Port=2
  FluxFlag : Inport  Port=3
  TorqueFlag : Inport  Port=4
  Flux : Inport  Port=5
  FluxRef : Inport  Port=6
  CenterSector : Sum
  FluxAddress : Gain  Gain=6
  FluxDirection : Trigonometry  Operator=atan2
  FullTurn : Constant  Value=2*pi  OutDataTypeStr=single
  HalfSector : Constant  Value=pi/6  OutDataTypeStr=single
  InitialVector : Constant  OutDataTypeStr=single
  PositiveDirection : Math  Operator=mod
  PrefluxRequired : RelationalOperator  Operator=<  OutDataTypeStr=boolean  RndMeth=Simplest  InputSameDT=off
  PrefluxThreshold : Gain  Gain=.80
  SectorBase : Constant  OutDataTypeStr=single
  SectorOneBased : Sum
  SectorZeroBased : Rounding
  SectorsPerRadian : Gain  Gain=3/pi
  StartupVector : Switch  Criteria=u2 ~= 0  SaturateOnIntegerOverflow=off  InputSameDT=off
  TableAddress : Sum  Inputs=+++
  TorqueAddress : Gain  Gain=12
  TorqueOffset : Constant  OutDataTypeStr=single
  TorqueRow : Sum
  UpperSwitchA : Lookup_n-D  NumberOfTableDimensions=1  BreakpointsForDimension1=single(0:7)  Table=single([0 1 1 0 0 0 1 1])  InterpMethod=Flat  ExtrapMethod=Clip  InternalRulePriority=Speed  RndMeth=Simplest
  UpperSwitchB : Lookup_n-D  NumberOfTableDimensions=1  BreakpointsForDimension1=single(0:7)  Table=single([0 0 1 1 1 0 0 1])  InterpMethod=Flat  ExtrapMethod=Clip  InternalRulePriority=Speed  RndMeth=Simplest
  UpperSwitchC : Lookup_n-D  NumberOfTableDimensions=1  BreakpointsForDimension1=single(0:7)  Table=single([0 0 0 0 1 1 1 1])  InterpMethod=Flat  ExtrapMethod=Clip  InternalRulePriority=Speed  RndMeth=Simplest
  VoltageVectorROM : Lookup_n-D  NumberOfTableDimensions=1  BreakpointsForDimension1=single(0:35)  Table=single([5 6 1 2 3 4 6 1 2 3 4 5 7 0 7 0 7 0 0 7 0 7 0 7 3 4 5 6 1 2 2 3 4 5 6 1])  InterpMethod=Flat  ExtrapMethod=Clip  InternalRulePriority=Speed  RndMeth=Simplest
  A : Outport
  B : Outport  Port=2
  C : Outport  Port=3
  SectorNumber : Outport  Port=4
  Index : Outport  Port=5
  wires:
  UpperSwitchC/1 -> C/1
  UpperSwitchB/1 -> B/1
  UpperSwitchA/1 -> A/1
  StartupVector/1 -> Index/1, UpperSwitchA/1, UpperSwitchB/1, UpperSwitchC/1
  VoltageVectorROM/1 -> StartupVector/3
  PrefluxRequired/1 -> StartupVector/2
  InitialVector/1 -> StartupVector/1
  PrefluxThreshold/1 -> PrefluxRequired/2
  Flux/1 -> PrefluxRequired/1
  FluxRef/1 -> PrefluxThreshold/1
  TableAddress/1 -> VoltageVectorROM/1
  TorqueAddress/1 -> TableAddress/3
  FluxAddress/1 -> TableAddress/2
  TorqueRow/1 -> TorqueAddress/1
  TorqueOffset/1 -> TorqueRow/2
  TorqueFlag/1 -> TorqueRow/1
  FluxFlag/1 -> FluxAddress/1
  SectorOneBased/1 -> SectorNumber/1
  SectorBase/1 -> SectorOneBased/2
  SectorZeroBased/1 -> SectorOneBased/1, TableAddress/1
  SectorsPerRadian/1 -> SectorZeroBased/1
  PositiveDirection/1 -> SectorsPerRadian/1
  FullTurn/1 -> PositiveDirection/2
  CenterSector/1 -> PositiveDirection/1
  HalfSector/1 -> CenterSector/2
  FluxDirection/1 -> CenterSector/1
  Alpha/1 -> FluxDirection/2
  Beta/1 -> FluxDirection/1

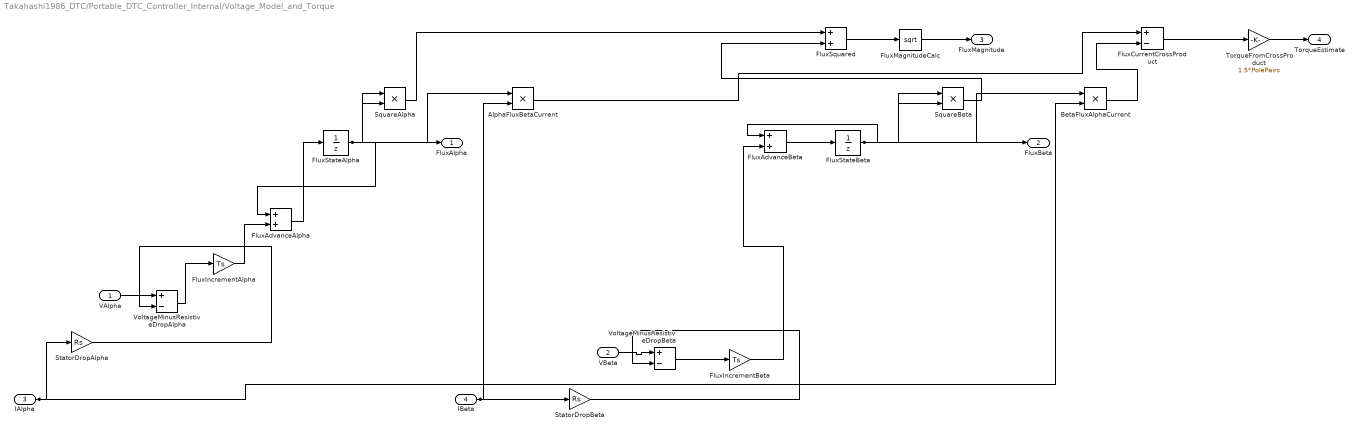
== system Takahashi1986_DTC/Portable_DTC_Controller_Internal/Voltage_Model_and_Torque ==
  VAlpha : Inport
  VBeta : Inport  Port=2
  IAlpha : Inport  Port=3
  IBeta : Inport  Port=4
  AlphaFluxBetaCurrent : Product  Inputs=**
  BetaFluxAlphaCurrent : Product  Inputs=**
  FluxAdvanceAlpha : Sum
  FluxAdvanceBeta : Sum
  FluxCurrentCrossProduct : Sum  Inputs=+-
  FluxIncrementAlpha : Gain  Gain=Ts
  FluxIncrementBeta : Gain  Gain=Ts
  FluxMagnitudeCalc : Sqrt
  FluxSquared : Sum
  FluxStateAlpha : UnitDelay  SampleTime=Ts  HasFrameUpgradeWarning=on
  FluxStateBeta : UnitDelay  SampleTime=Ts  HasFrameUpgradeWarning=on
  SquareAlpha : Product  Inputs=**
  SquareBeta : Product  Inputs=**
  StatorDropAlpha : Gain  Gain=Rs
  StatorDropBeta : Gain  Gain=Rs
  TorqueFromCrossProduct : Gain  Gain=1.5*PolePairs
  VoltageMinusResistiveDropAlpha : Sum  Inputs=+-
  VoltageMinusResistiveDropBeta : Sum  Inputs=+-
  FluxAlpha : Outport
  FluxBeta : Outport  Port=2
  FluxMagnitude : Outport  Port=3
  TorqueEstimate : Outport  Port=4
  wires:
  TorqueFromCrossProduct/1 -> TorqueEstimate/1
  FluxCurrentCrossProduct/1 -> TorqueFromCrossProduct/1
  BetaFluxAlphaCurrent/1 -> FluxCurrentCrossProduct/2
  AlphaFluxBetaCurrent/1 -> FluxCurrentCrossProduct/1
  FluxMagnitudeCalc/1 -> FluxMagnitude/1
  FluxSquared/1 -> FluxMagnitudeCalc/1
  SquareBeta/1 -> FluxSquared/2
  SquareAlpha/1 -> FluxSquared/1
  FluxAdvanceBeta/1 -> FluxStateBeta/1
  FluxIncrementBeta/1 -> FluxAdvanceBeta/2
  FluxStateBeta/1 -> FluxAdvanceBeta/1, FluxBeta/1, BetaFluxAlphaCurrent/1, SquareBeta/1, SquareBeta/2
  VoltageMinusResistiveDropBeta/1 -> FluxIncrementBeta/1
  StatorDropBeta/1 -> VoltageMinusResistiveDropBeta/2
  VBeta/1 -> VoltageMinusResistiveDropBeta/1
  IBeta/1 -> StatorDropBeta/1, AlphaFluxBetaCurrent/2
  FluxAdvanceAlpha/1 -> FluxStateAlpha/1
  FluxIncrementAlpha/1 -> FluxAdvanceAlpha/2
  FluxStateAlpha/1 -> FluxAdvanceAlpha/1, FluxAlpha/1, AlphaFluxBetaCurrent/1, SquareAlpha/1, SquareAlpha/2
  VoltageMinusResistiveDropAlpha/1 -> FluxIncrementAlpha/1
  StatorDropAlpha/1 -> VoltageMinusResistiveDropAlpha/2
  VAlpha/1 -> VoltageMinusResistiveDropAlpha/1
  IAlpha/1 -> BetaFluxAlphaCurrent/2, StatorDropAlpha/1
